simulink model "mod_am"  (R2024b)
settings: Solver=FixedStepDiscrete  StartTime=0.0  StopTime=0.05  FixedStep=5e-06  RelTol=1e-3
model workspace (MAT data in the model file):
  fc = 10000
  fm = 1000
  fs = 200000
  hpre = [-9.37676366463e-20 -1.20782423708e-05 -2.42221352139e-05 -3.6375450657e-05 -4.84796495276e-05 -6.04732906365e-05 -7.22914850986e-05 -8.38654166577e-05 -9.51219482678e-05 -0.000105983334092 -0.000116367054612 -0.00012618579071 ... (401 elements, 1x401)]
  m = 0.5
  phi = 0.7
  sigma2 = 0.02
settings Model: Creator=runner  LastModifiedBy=runner

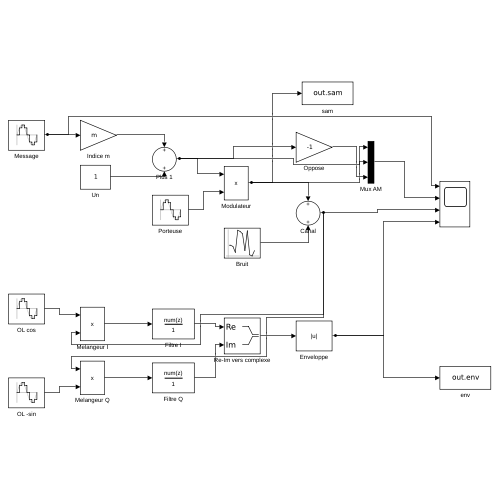
[thumbnail: Simulink's stored preview of the top-level diagram]
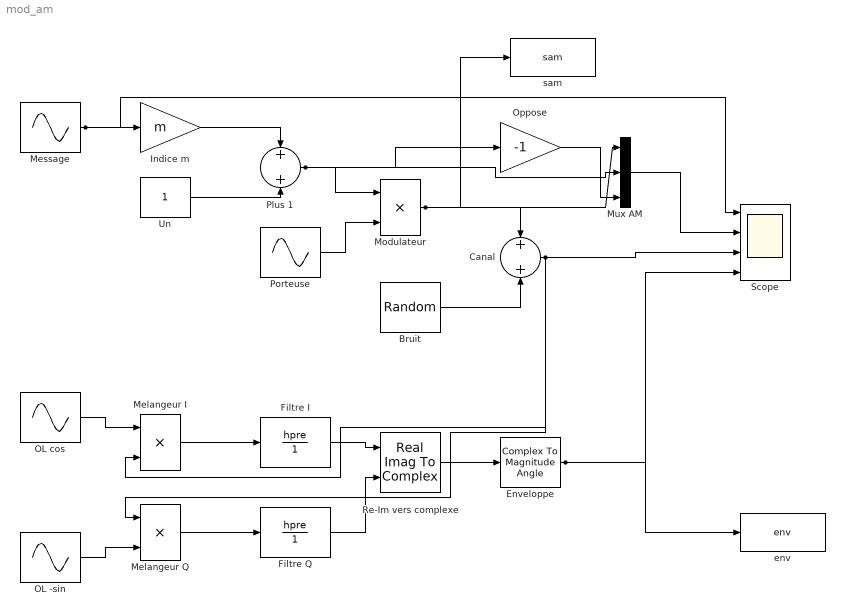
== system mod_am ==
  Bruit : RandomNumber  Variance=sigma2  Seed=1  SampleTime=1/fs
  Canal : Sum
  Enveloppe : ComplexToMagnitudeAngle  Output=Magnitude
  Filtre I : DiscreteFilter  Numerator=hpre  Denominator=1
  Filtre Q : DiscreteFilter  Numerator=hpre  Denominator=1
  Indice m : Gain  Gain=m
  Melangeur I : Product
  Melangeur Q : Product
  Message : Sin  Frequency=2*pi*fm  Phase=pi/2  SampleTime=1/fs
  Modulateur : Product
  Mux AM : Mux  Inputs=3
  OL -sin : Sin  Amplitude=-2  Frequency=2*pi*fc  SampleTime=1/fs
  OL cos : Sin  Amplitude=2  Frequency=2*pi*fc  Phase=pi/2  SampleTime=1/fs
  Oppose : Gain  Gain=-1
  Plus 1 : Sum
  Porteuse : Sin  Frequency=2*pi*fc  Phase=pi/2+phi  SampleTime=1/fs
  Re-Im vers complexe : RealImagToComplex
  Scope : Scope  NumInputPorts=4
  Un : Constant
  env : ToWorkspace  VariableName=env  SampleTime=-1
  sam : ToWorkspace  VariableName=sam  SampleTime=-1
  wires:
  Message/1 -> Indice m/1, Scope/1
  Indice m/1 -> Plus 1/1
  Un/1 -> Plus 1/2
  Plus 1/1 -> Modulateur/1, Oppose/1, Mux AM/2
  Porteuse/1 -> Modulateur/2
  Modulateur/1 -> Canal/1, Mux AM/1, sam/1
  Bruit/1 -> Canal/2
  Oppose/1 -> Mux AM/3
  OL cos/1 -> Melangeur I/1
  Canal/1 -> Melangeur I/2, Melangeur Q/1, Scope/3
  OL -sin/1 -> Melangeur Q/2
  Melangeur I/1 -> Filtre I/1
  Melangeur Q/1 -> Filtre Q/1
  Filtre I/1 -> Re-Im vers complexe/1
  Filtre Q/1 -> Re-Im vers complexe/2
  Re-Im vers complexe/1 -> Enveloppe/1
  Enveloppe/1 -> env/1, Scope/4
  Mux AM/1 -> Scope/2
